simulink model "Prey_Predator_STM32F4"  (R2025a)
settings: Solver=FixedStepDiscrete  StartTime=0.0  StopTime=10.0  RelTol=1e-3
PreLoadFcn:
  | waijung.modelPreload; % Required for working with Waijung Blockset. Do not remove.
undefined symbols (not defined in the file): HSEOSC, Link, LQFP176, ST, STM32F417IG
libraries: stm32f4_io_lib x144, fuzblock x1, stm32f4_device_config_lib x1
(part 2 of 3)

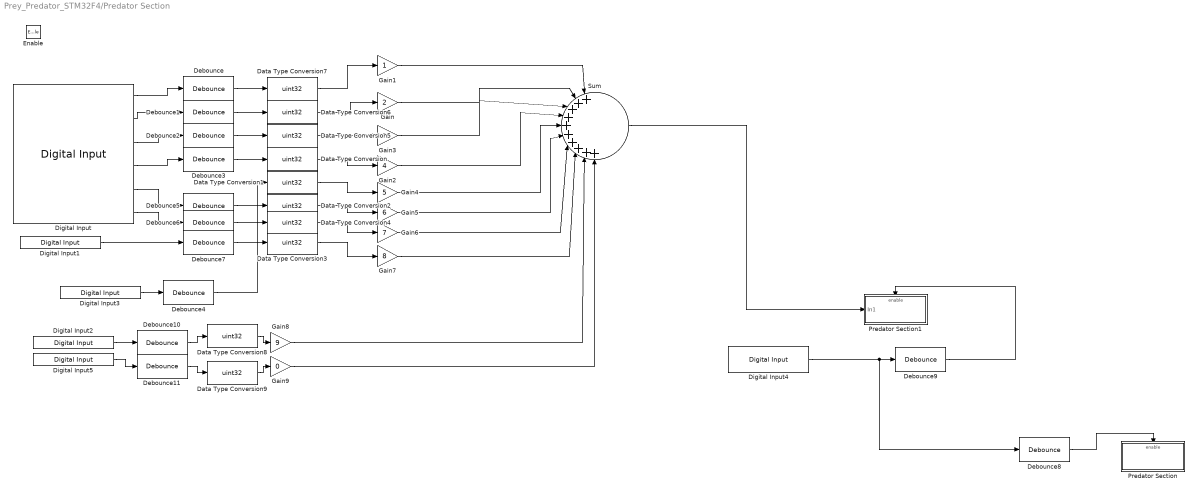
== system Prey_Predator_STM32F4/Predator Section ==
  Enable : EnablePort  PropagateVarSize=During execution
  Data Type Conversion{,1..9} (10 alike) : DataTypeConversion  OutDataTypeStr=uint32  SaturateOnIntegerOverflow=off  RndMeth=Floor
  Debounce{,1..8,10..11} (11 alike) : stm32f4_io_lib/Debounce  mode=Normal  prescale=4  debounce=4
      settings: SourceProductName=IO
  Debounce9 : stm32f4_io_lib/Debounce  mode=Single Pulse  prescale=4  debounce=4
      settings: SourceProductName=IO
  Digital Input : stm32f4_io_lib/Digital Input  port=D  speed=100  porttype=None  porttypestr=NOPULL  use_pin0=off  use_pin1=on  use_pin2=on  use_pin3=on  use_pin4=on  use_pin5=off  use_pin6=on  use_pin7=on  use_pin8=off  use_pin9=off  use_pin10=off  use_pin11=off  use_pin12=off  use_pin13=off  use_pin14=off  use_pin15=off  pinstr=GPIO_Pin_1 | GPIO_Pin_2 | GPIO_Pin_3 | GPIO_Pin_4 | GPIO_Pin_6 | GPIO_Pin_7  usedpinarray="[0  1  1  1  1  0  1  1  0  0  0  0  0  0  0  0]"  bitbandingstr=|  sampletime=0.01  sampletimestr=-1  blockid=PredatorSectionDigitalInput  enablecustomportlabel=off  glabalinit=off  cinputportlabel=In1, In2  coutputportlabel=Out1, Out2
      | #define PredatorSectionDigitalInput_D1 Peripheral_BB(GPIOD->IDR, 1)  /* Output pin */
      | #define PredatorSectionDigitalInput_D2 Peripheral_BB(GPIOD->IDR, 2)  /* Output pin */
      | #define PredatorSectionDigitalInput_D3 Peripheral_BB(GPIOD->IDR, 3)  /* Output pin */
      | #define PredatorSectionDigitalInput_D4 Peripheral_BB(GPIOD->IDR, 4)  /* Output pin */
      | #define PredatorSectionDigitalInput_D6 Peripheral_BB(GPIOD->IDR, 6)  /* Output pin */
      | #define PredatorSectionDigitalInput_D7 Peripheral_BB(GPIOD->IDR, 7)  /* Output pin */
      settings: SourceProductName=IO
  Digital Input1 : stm32f4_io_lib/Digital Input  port=B  speed=100  porttype=None  porttypestr=NOPULL  use_pin0=off  use_pin1=off  use_pin2=off  use_pin3=on  use_pin4=off  use_pin5=off  use_pin6=off  use_pin7=off  use_pin8=off  use_pin9=off  use_pin10=off  use_pin11=off  use_pin12=off  use_pin13=off  use_pin14=off  use_pin15=off  pinstr=GPIO_Pin_3  usedpinarray="[0  0  0  1  0  0  0  0  0  0  0  0  0  0  0  0]"  bitbandingstr="#define PredatorSectionDigitalInput1_B3 Peripheral_BB(GPIOB->IDR, 3)  /* Output pin */"  sampletime=0.01  sampletimestr=-1  blockid=PredatorSectionDigitalInput1  enablecustomportlabel=off  glabalinit=off  cinputportlabel=In1, In2  coutputportlabel=Out1, Out2
      settings: SourceProductName=IO
  Digital Input2 : stm32f4_io_lib/Digital Input  port=A  speed=100  porttype=None  porttypestr=NOPULL  use_pin0=off  use_pin1=on  use_pin2=off  use_pin3=off  use_pin4=off  use_pin5=off  use_pin6=off  use_pin7=off  use_pin8=off  use_pin9=off  use_pin10=off  use_pin11=off  use_pin12=off  use_pin13=off  use_pin14=off  use_pin15=off  pinstr=GPIO_Pin_1  usedpinarray="[0  1  0  0  0  0  0  0  0  0  0  0  0  0  0  0]"  bitbandingstr="#define PredatorSectionDigitalInput2_A1 Peripheral_BB(GPIOA->IDR, 1)  /* Output pin */"  sampletime=0.01  sampletimestr=-1  blockid=PredatorSectionDigitalInput2  enablecustomportlabel=off  glabalinit=off  cinputportlabel=In1, In2  coutputportlabel=Out1, Out2
      settings: SourceProductName=IO
  Digital Input3 : stm32f4_io_lib/Digital Input  port=B  speed=100  porttype=None  porttypestr=NOPULL  use_pin0=off  use_pin1=off  use_pin2=off  use_pin3=off  use_pin4=off  use_pin5=on  use_pin6=off  use_pin7=off  use_pin8=off  use_pin9=off  use_pin10=off  use_pin11=off  use_pin12=off  use_pin13=off  use_pin14=off  use_pin15=off  pinstr=GPIO_Pin_5  usedpinarray="[0  0  0  0  0  1  0  0  0  0  0  0  0  0  0  0]"  bitbandingstr="#define PredatorSectionDigitalInput3_B5 Peripheral_BB(GPIOB->IDR, 5)  /* Output pin */"  sampletime=0.01  sampletimestr=-1  blockid=PredatorSectionDigitalInput3  enablecustomportlabel=off  glabalinit=off  cinputportlabel=In1, In2  coutputportlabel=Out1, Out2
      settings: SourceProductName=IO
  Digital Input4 : stm32f4_io_lib/Digital Input  port=E  speed=100  porttype=None  porttypestr=NOPULL  use_pin0=off  use_pin1=off  use_pin2=on  use_pin3=off  use_pin4=off  use_pin5=off  use_pin6=off  use_pin7=off  use_pin8=off  use_pin9=off  use_pin10=off  use_pin11=off  use_pin12=off  use_pin13=off  use_pin14=off  use_pin15=off  pinstr=GPIO_Pin_2  usedpinarray="[0  0  1  0  0  0  0  0  0  0  0  0  0  0  0  0]"  bitbandingstr="#define PredatorSectionDigitalInput4_E2 Peripheral_BB(GPIOE->IDR, 2)  /* Output pin */"  sampletime=0.01  sampletimestr=-1  blockid=PredatorSectionDigitalInput4  enablecustomportlabel=off  glabalinit=off  cinputportlabel=In1, In2  coutputportlabel=Out1, Out2
      settings: SourceProductName=IO
  Digital Input5 : stm32f4_io_lib/Digital Input  port=A  speed=100  porttype=None  porttypestr=NOPULL  use_pin0=on  use_pin1=off  use_pin2=off  use_pin3=off  use_pin4=off  use_pin5=off  use_pin6=off  use_pin7=off  use_pin8=off  use_pin9=off  use_pin10=off  use_pin11=off  use_pin12=off  use_pin13=off  use_pin14=off  use_pin15=off  pinstr=GPIO_Pin_0  usedpinarray="[1  0  0  0  0  0  0  0  0  0  0  0  0  0  0  0]"  bitbandingstr="#define PredatorSectionDigitalInput5_A0 Peripheral_BB(GPIOA->IDR, 0)  /* Output pin */"  sampletime=0.01  sampletimestr=-1  blockid=PredatorSectionDigitalInput5  enablecustomportlabel=off  glabalinit=off  cinputportlabel=In1, In2  coutputportlabel=Out1, Out2
      settings: SourceProductName=IO
  Gain : Gain  Gain=2  OutDataTypeStr=Inherit: Same as input
  Gain1 : Gain  OutDataTypeStr=Inherit: Same as input
  Gain2 : Gain  Gain=4  OutDataTypeStr=Inherit: Same as input
  Gain3 : Gain  Gain=3  OutDataTypeStr=Inherit: Same as input
  Gain4 : Gain  Gain=5  OutDataTypeStr=Inherit: Same as input
  Gain5 : Gain  Gain=6  OutDataTypeStr=Inherit: Same as input
  Gain6 : Gain  Gain=7  OutDataTypeStr=Inherit: Same as input
  Gain7 : Gain  Gain=8  OutDataTypeStr=Inherit: Same as input
  Gain8 : Gain  Gain=9  OutDataTypeStr=Inherit: Same as input
  Gain9 : Gain  Gain=0  OutDataTypeStr=Inherit: Same as input
  Predator Section : Subsystem
  Predator Section1 : Subsystem
  Sum : Sum  Inputs=|++++++++++
  wires:
  Digital Input/4 -> Debounce3/1
  Digital Input/3 -> Debounce2/1
  Digital Input/2 -> Debounce1/1
  Digital Input/1 -> Debounce/1
  Digital Input1/1 -> Debounce7/1
  Debounce/1 -> Data Type Conversion7/1
  Debounce1/1 -> Data Type Conversion6/1
  Debounce2/1 -> Data Type Conversion5/1
  Debounce3/1 -> Data Type Conversion/1
  Debounce4/1 -> Data Type Conversion1/1
  Debounce5/1 -> Data Type Conversion2/1
  Debounce6/1 -> Data Type Conversion4/1
  Debounce7/1 -> Data Type Conversion3/1
  Data Type Conversion7/1 -> Gain1/1
  Data Type Conversion6/1 -> Gain/1
  Data Type Conversion5/1 -> Gain3/1
  Data Type Conversion/1 -> Gain2/1
  Data Type Conversion1/1 -> Gain4/1
  Data Type Conversion2/1 -> Gain5/1
  Data Type Conversion4/1 -> Gain6/1
  Data Type Conversion3/1 -> Gain7/1
  Gain1/1 -> Sum/1
  Gain/1 -> Sum/2
  Gain3/1 -> Sum/3
  Gain2/1 -> Sum/4
  Gain4/1 -> Sum/5
  Gain5/1 -> Sum/6
  Gain6/1 -> Sum/7
  Gain7/1 -> Sum/8
  Digital Input/5 -> Debounce5/1
  Digital Input/6 -> Debounce6/1
  Digital Input3/1 -> Debounce4/1
  Sum/1 -> Predator Section1/1(In1)
  Digital Input4/1 -> Debounce8/1, Debounce9/1
  Debounce9/1 -> Predator Section1/Enable
  Debounce8/1 -> Predator Section/Enable
  Digital Input2/1 -> Debounce10/1
  Digital Input5/1 -> Debounce11/1
  Debounce11/1 -> Data Type Conversion9/1
  Debounce10/1 -> Data Type Conversion8/1
  Data Type Conversion8/1 -> Gain8/1
  Data Type Conversion9/1 -> Gain9/1
  Gain8/1 -> Sum/9
  Gain9/1 -> Sum/10

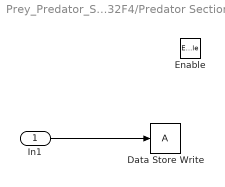
== system Prey_Predator_STM32F4/Predator Section1 ==
  In1 : Inport
  Enable : EnablePort  PropagateVarSize=During execution
  Data Store Write : DataStoreWrite  IndexOptions=Index vector (dialog)  Indices=1  OutputSizes=1
  wires:
  In1/1 -> Data Store Write/1

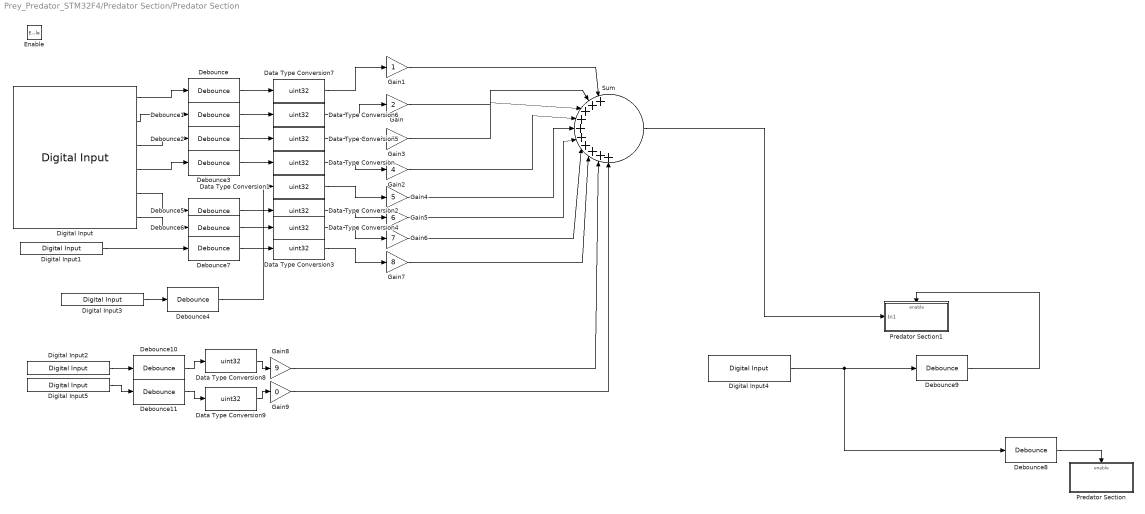
== system Prey_Predator_STM32F4/Predator Section/Predator Section ==
  Enable : EnablePort  PropagateVarSize=During execution
  Data Type Conversion{,1..9} (10 alike) : DataTypeConversion  OutDataTypeStr=uint32  SaturateOnIntegerOverflow=off  RndMeth=Floor
  Debounce{,1..8,10..11} (11 alike) : stm32f4_io_lib/Debounce  mode=Normal  prescale=4  debounce=4
      settings: SourceProductName=IO
  Debounce9 : stm32f4_io_lib/Debounce  mode=Single Pulse  prescale=4  debounce=4
      settings: SourceProductName=IO
  Digital Input : stm32f4_io_lib/Digital Input  port=D  speed=100  porttype=None  porttypestr=NOPULL  use_pin0=off  use_pin1=on  use_pin2=on  use_pin3=on  use_pin4=on  use_pin5=off  use_pin6=on  use_pin7=on  use_pin8=off  use_pin9=off  use_pin10=off  use_pin11=off  use_pin12=off  use_pin13=off  use_pin14=off  use_pin15=off  pinstr=GPIO_Pin_1 | GPIO_Pin_2 | GPIO_Pin_3 | GPIO_Pin_4 | GPIO_Pin_6 | GPIO_Pin_7  usedpinarray="[0  1  1  1  1  0  1  1  0  0  0  0  0  0  0  0]"  bitbandingstr=|  sampletime=0.01  sampletimestr=-1  blockid=PredatorSectionPredatorSectionDigitalInput  enablecustomportlabel=off  glabalinit=off  cinputportlabel=In1, In2  coutputportlabel=Out1, Out2
      | #define PredatorSectionPredatorSectionDigitalInput_D1 Peripheral_BB(GPIOD->IDR, 1)  /* Output pin */
      | #define PredatorSectionPredatorSectionDigitalInput_D2 Peripheral_BB(GPIOD->IDR, 2)  /* Output pin */
      | #define PredatorSectionPredatorSectionDigitalInput_D3 Peripheral_BB(GPIOD->IDR, 3)  /* Output pin */
      | #define PredatorSectionPredatorSectionDigitalInput_D4 Peripheral_BB(GPIOD->IDR, 4)  /* Output pin */
      | #define PredatorSectionPredatorSectionDigitalInput_D6 Peripheral_BB(GPIOD->IDR, 6)  /* Output pin */
      | #define PredatorSectionPredatorSectionDigitalInput_D7 Peripheral_BB(GPIOD->IDR, 7)  /* Output pin */
      settings: SourceProductName=IO
  Digital Input1 : stm32f4_io_lib/Digital Input  port=B  speed=100  porttype=None  porttypestr=NOPULL  use_pin0=off  use_pin1=off  use_pin2=off  use_pin3=on  use_pin4=off  use_pin5=off  use_pin6=off  use_pin7=off  use_pin8=off  use_pin9=off  use_pin10=off  use_pin11=off  use_pin12=off  use_pin13=off  use_pin14=off  use_pin15=off  pinstr=GPIO_Pin_3  usedpinarray="[0  0  0  1  0  0  0  0  0  0  0  0  0  0  0  0]"  bitbandingstr="#define PredatorSectionPredatorSectionDigitalInput1_B3 Peripheral_BB(GPIOB->IDR, 3)  /* Output pin */"  sampletime=0.01  sampletimestr=-1  blockid=PredatorSectionPredatorSectionDigitalInput1  enablecustomportlabel=off  glabalinit=off  cinputportlabel=In1, In2  coutputportlabel=Out1, Out2
      settings: SourceProductName=IO
  Digital Input2 : stm32f4_io_lib/Digital Input  port=A  speed=100  porttype=None  porttypestr=NOPULL  use_pin0=off  use_pin1=on  use_pin2=off  use_pin3=off  use_pin4=off  use_pin5=off  use_pin6=off  use_pin7=off  use_pin8=off  use_pin9=off  use_pin10=off  use_pin11=off  use_pin12=off  use_pin13=off  use_pin14=off  use_pin15=off  pinstr=GPIO_Pin_1  usedpinarray="[0  1  0  0  0  0  0  0  0  0  0  0  0  0  0  0]"  bitbandingstr="#define PredatorSectionPredatorSectionDigitalInput2_A1 Peripheral_BB(GPIOA->IDR, 1)  /* Output pin */"  sampletime=0.01  sampletimestr=-1  blockid=PredatorSectionPredatorSectionDigitalInput2  enablecustomportlabel=off  glabalinit=off  cinputportlabel=In1, In2  coutputportlabel=Out1, Out2
      settings: SourceProductName=IO
  Digital Input3 : stm32f4_io_lib/Digital Input  port=B  speed=100  porttype=None  porttypestr=NOPULL  use_pin0=off  use_pin1=off  use_pin2=off  use_pin3=off  use_pin4=off  use_pin5=on  use_pin6=off  use_pin7=off  use_pin8=off  use_pin9=off  use_pin10=off  use_pin11=off  use_pin12=off  use_pin13=off  use_pin14=off  use_pin15=off  pinstr=GPIO_Pin_5  usedpinarray="[0  0  0  0  0  1  0  0  0  0  0  0  0  0  0  0]"  bitbandingstr="#define PredatorSectionPredatorSectionDigitalInput3_B5 Peripheral_BB(GPIOB->IDR, 5)  /* Output pin */"  sampletime=0.01  sampletimestr=-1  blockid=PredatorSectionPredatorSectionDigitalInput3  enablecustomportlabel=off  glabalinit=off  cinputportlabel=In1, In2  coutputportlabel=Out1, Out2
      settings: SourceProductName=IO
  Digital Input4 : stm32f4_io_lib/Digital Input  port=A  speed=100  porttype=None  porttypestr=NOPULL  use_pin0=off  use_pin1=off  use_pin2=off  use_pin3=off  use_pin4=off  use_pin5=off  use_pin6=off  use_pin7=off  use_pin8=off  use_pin9=off  use_pin10=off  use_pin11=off  use_pin12=off  use_pin13=off  use_pin14=off  use_pin15=on  pinstr=GPIO_Pin_15  usedpinarray="[0  0  0  0  0  0  0  0  0  0  0  0  0  0  0  1]"  bitbandingstr="#define PredatorSectionPredatorSectionDigitalInput4_A15 Peripheral_BB(GPIOA->IDR, 15)  /* Output pin */"  sampletime=0.01  sampletimestr=-1  blockid=PredatorSectionPredatorSectionDigitalInput4  enablecustomportlabel=off  glabalinit=off  cinputportlabel=In1, In2  coutputportlabel=Out1, Out2
      settings: SourceProductName=IO
  Digital Input5 : stm32f4_io_lib/Digital Input  port=A  speed=100  porttype=None  porttypestr=NOPULL  use_pin0=on  use_pin1=off  use_pin2=off  use_pin3=off  use_pin4=off  use_pin5=off  use_pin6=off  use_pin7=off  use_pin8=off  use_pin9=off  use_pin10=off  use_pin11=off  use_pin12=off  use_pin13=off  use_pin14=off  use_pin15=off  pinstr=GPIO_Pin_0  usedpinarray="[1  0  0  0  0  0  0  0  0  0  0  0  0  0  0  0]"  bitbandingstr="#define PredatorSectionPredatorSectionDigitalInput5_A0 Peripheral_BB(GPIOA->IDR, 0)  /* Output pin */"  sampletime=0.01  sampletimestr=-1  blockid=PredatorSectionPredatorSectionDigitalInput5  enablecustomportlabel=off  glabalinit=off  cinputportlabel=In1, In2  coutputportlabel=Out1, Out2
      settings: SourceProductName=IO
  Gain : Gain  Gain=2  OutDataTypeStr=Inherit: Same as input
  Gain1 : Gain  OutDataTypeStr=Inherit: Same as input
  Gain2 : Gain  Gain=4  OutDataTypeStr=Inherit: Same as input
  Gain3 : Gain  Gain=3  OutDataTypeStr=Inherit: Same as input
  Gain4 : Gain  Gain=5  OutDataTypeStr=Inherit: Same as input
  Gain5 : Gain  Gain=6  OutDataTypeStr=Inherit: Same as input
  Gain6 : Gain  Gain=7  OutDataTypeStr=Inherit: Same as input
  Gain7 : Gain  Gain=8  OutDataTypeStr=Inherit: Same as input
  Gain8 : Gain  Gain=9  OutDataTypeStr=Inherit: Same as input
  Gain9 : Gain  Gain=0  OutDataTypeStr=Inherit: Same as input
  Predator Section : Subsystem
  Predator Section1 : Subsystem
  Sum : Sum  Inputs=|++++++++++
  wires:
  Digital Input/4 -> Debounce3/1
  Digital Input/3 -> Debounce2/1
  Digital Input/2 -> Debounce1/1
  Digital Input/1 -> Debounce/1
  Digital Input1/1 -> Debounce7/1
  Debounce/1 -> Data Type Conversion7/1
  Debounce1/1 -> Data Type Conversion6/1
  Debounce2/1 -> Data Type Conversion5/1
  Debounce3/1 -> Data Type Conversion/1
  Debounce4/1 -> Data Type Conversion1/1
  Debounce5/1 -> Data Type Conversion2/1
  Debounce6/1 -> Data Type Conversion4/1
  Debounce7/1 -> Data Type Conversion3/1
  Data Type Conversion7/1 -> Gain1/1
  Data Type Conversion6/1 -> Gain/1
  Data Type Conversion5/1 -> Gain3/1
  Data Type Conversion/1 -> Gain2/1
  Data Type Conversion1/1 -> Gain4/1
  Data Type Conversion2/1 -> Gain5/1
  Data Type Conversion4/1 -> Gain6/1
  Data Type Conversion3/1 -> Gain7/1
  Gain1/1 -> Sum/1
  Gain/1 -> Sum/2
  Gain3/1 -> Sum/3
  Gain2/1 -> Sum/4
  Gain4/1 -> Sum/5
  Gain5/1 -> Sum/6
  Gain6/1 -> Sum/7
  Gain7/1 -> Sum/8
  Digital Input/5 -> Debounce5/1
  Digital Input/6 -> Debounce6/1
  Digital Input3/1 -> Debounce4/1
  Sum/1 -> Predator Section1/1(In1)
  Digital Input4/1 -> Debounce8/1, Debounce9/1
  Debounce9/1 -> Predator Section1/Enable
  Debounce8/1 -> Predator Section/Enable
  Digital Input2/1 -> Debounce10/1
  Digital Input5/1 -> Debounce11/1
  Debounce11/1 -> Data Type Conversion9/1
  Debounce10/1 -> Data Type Conversion8/1
  Data Type Conversion8/1 -> Gain8/1
  Data Type Conversion9/1 -> Gain9/1
  Gain8/1 -> Sum/9
  Gain9/1 -> Sum/10

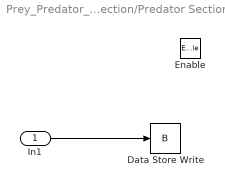
== system Prey_Predator_STM32F4/Predator Section/Predator Section1 ==
  In1 : Inport
  Enable : EnablePort  PropagateVarSize=During execution
  Data Store Write : DataStoreWrite  DataStoreName=B  IndexOptions=Index vector (dialog)  Indices=1  OutputSizes=1
  wires:
  In1/1 -> Data Store Write/1

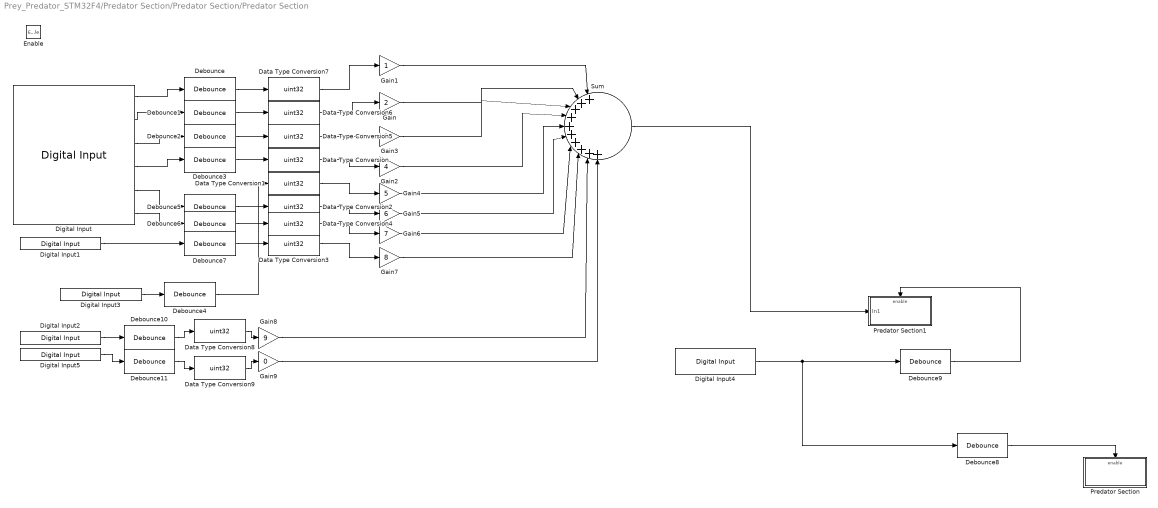
== system Prey_Predator_STM32F4/Predator Section/Predator Section/Predator Section ==
  Enable : EnablePort  PropagateVarSize=During execution
  Data Type Conversion{,1..9} (10 alike) : DataTypeConversion  OutDataTypeStr=uint32  SaturateOnIntegerOverflow=off  RndMeth=Floor
  Debounce{,1..8,10..11} (11 alike) : stm32f4_io_lib/Debounce  mode=Normal  prescale=4  debounce=4
      settings: SourceProductName=IO
  Debounce9 : stm32f4_io_lib/Debounce  mode=Single Pulse  prescale=4  debounce=4
      settings: SourceProductName=IO
  Digital Input : stm32f4_io_lib/Digital Input  port=D  speed=100  porttype=None  porttypestr=NOPULL  use_pin0=off  use_pin1=on  use_pin2=on  use_pin3=on  use_pin4=on  use_pin5=off  use_pin6=on  use_pin7=on  use_pin8=off  use_pin9=off  use_pin10=off  use_pin11=off  use_pin12=off  use_pin13=off  use_pin14=off  use_pin15=off  pinstr=GPIO_Pin_1 | GPIO_Pin_2 | GPIO_Pin_3 | GPIO_Pin_4 | GPIO_Pin_6 | GPIO_Pin_7  usedpinarray="[0  1  1  1  1  0  1  1  0  0  0  0  0  0  0  0]"  bitbandingstr=|  sampletime=0.01  sampletimestr=-1  blockid=PredatorSectionPredatorSectionPredatorSectionDigitalInput  enablecustomportlabel=off  glabalinit=off  cinputportlabel=In1, In2  coutputportlabel=Out1, Out2
      | #define PredatorSectionPredatorSectionPredatorSectionDigitalInput_D1 Peripheral_BB(GPIOD->IDR, 1)  /* Output pin */
      | #define PredatorSectionPredatorSectionPredatorSectionDigitalInput_D2 Peripheral_BB(GPIOD->IDR, 2)  /* Output pin */
      | #define PredatorSectionPredatorSectionPredatorSectionDigitalInput_D3 Peripheral_BB(GPIOD->IDR, 3)  /* Output pin */
      | #define PredatorSectionPredatorSectionPredatorSectionDigitalInput_D4 Peripheral_BB(GPIOD->IDR, 4)  /* Output pin */
      | #define PredatorSectionPredatorSectionPredatorSectionDigitalInput_D6 Peripheral_BB(GPIOD->IDR, 6)  /* Output pin */
      | #define PredatorSectionPredatorSectionPredatorSectionDigitalInput_D7 Peripheral_BB(GPIOD->IDR, 7)  /* Output pin */
      settings: SourceProductName=IO
  Digital Input1 : stm32f4_io_lib/Digital Input  port=B  speed=100  porttype=None  porttypestr=NOPULL  use_pin0=off  use_pin1=off  use_pin2=off  use_pin3=on  use_pin4=off  use_pin5=off  use_pin6=off  use_pin7=off  use_pin8=off  use_pin9=off  use_pin10=off  use_pin11=off  use_pin12=off  use_pin13=off  use_pin14=off  use_pin15=off  pinstr=GPIO_Pin_3  usedpinarray="[0  0  0  1  0  0  0  0  0  0  0  0  0  0  0  0]"  bitbandingstr="#define PredatorSectionPredatorSectionPredatorSectionDigitalInput1_B3 Peripheral_BB(GPIOB->IDR, 3)  /* Output pin */"  sampletime=0.01  sampletimestr=-1  blockid=PredatorSectionPredatorSectionPredatorSectionDigitalInput1  enablecustomportlabel=off  glabalinit=off  cinputportlabel=In1, In2  coutputportlabel=Out1, Out2
      settings: SourceProductName=IO
  Digital Input2 : stm32f4_io_lib/Digital Input  port=A  speed=100  porttype=None  porttypestr=NOPULL  use_pin0=off  use_pin1=on  use_pin2=off  use_pin3=off  use_pin4=off  use_pin5=off  use_pin6=off  use_pin7=off  use_pin8=off  use_pin9=off  use_pin10=off  use_pin11=off  use_pin12=off  use_pin13=off  use_pin14=off  use_pin15=off  pinstr=GPIO_Pin_1  usedpinarray="[0  1  0  0  0  0  0  0  0  0  0  0  0  0  0  0]"  bitbandingstr="#define PredatorSectionPredatorSectionPredatorSectionDigitalInput2_A1 Peripheral_BB(GPIOA->IDR, 1)  /* Output pin */"  sampletime=0.01  sampletimestr=-1  blockid=PredatorSectionPredatorSectionPredatorSectionDigitalInput2  enablecustomportlabel=off  glabalinit=off  cinputportlabel=In1, In2  coutputportlabel=Out1, Out2
      settings: SourceProductName=IO
  Digital Input3 : stm32f4_io_lib/Digital Input  port=B  speed=100  porttype=None  porttypestr=NOPULL  use_pin0=off  use_pin1=off  use_pin2=off  use_pin3=off  use_pin4=off  use_pin5=on  use_pin6=off  use_pin7=off  use_pin8=off  use_pin9=off  use_pin10=off  use_pin11=off  use_pin12=off  use_pin13=off  use_pin14=off  use_pin15=off  pinstr=GPIO_Pin_5  usedpinarray="[0  0  0  0  0  1  0  0  0  0  0  0  0  0  0  0]"  bitbandingstr="#define PredatorSectionPredatorSectionPredatorSectionDigitalInput3_B5 Peripheral_BB(GPIOB->IDR, 5)  /* Output pin */"  sampletime=0.01  sampletimestr=-1  blockid=PredatorSectionPredatorSectionPredatorSectionDigitalInput3  enablecustomportlabel=off  glabalinit=off  cinputportlabel=In1, In2  coutputportlabel=Out1, Out2
      settings: SourceProductName=IO
  Digital Input4 : stm32f4_io_lib/Digital Input  port=E  speed=100  porttype=None  porttypestr=NOPULL  use_pin0=off  use_pin1=off  use_pin2=off  use_pin3=off  use_pin4=on  use_pin5=off  use_pin6=off  use_pin7=off  use_pin8=off  use_pin9=off  use_pin10=off  use_pin11=off  use_pin12=off  use_pin13=off  use_pin14=off  use_pin15=off  pinstr=GPIO_Pin_4  usedpinarray="[0  0  0  0  1  0  0  0  0  0  0  0  0  0  0  0]"  bitbandingstr="#define PredatorSectionPredatorSectionPredatorSectionDigitalInput4_E4 Peripheral_BB(GPIOE->IDR, 4)  /* Output pin */"  sampletime=0.01  sampletimestr=-1  blockid=PredatorSectionPredatorSectionPredatorSectionDigitalInput4  enablecustomportlabel=off  glabalinit=off  cinputportlabel=In1, In2  coutputportlabel=Out1, Out2
      settings: SourceProductName=IO
  Digital Input5 : stm32f4_io_lib/Digital Input  port=A  speed=100  porttype=None  porttypestr=NOPULL  use_pin0=on  use_pin1=off  use_pin2=off  use_pin3=off  use_pin4=off  use_pin5=off  use_pin6=off  use_pin7=off  use_pin8=off  use_pin9=off  use_pin10=off  use_pin11=off  use_pin12=off  use_pin13=off  use_pin14=off  use_pin15=off  pinstr=GPIO_Pin_0  usedpinarray="[1  0  0  0  0  0  0  0  0  0  0  0  0  0  0  0]"  bitbandingstr="#define PredatorSectionPredatorSectionPredatorSectionDigitalInput5_A0 Peripheral_BB(GPIOA->IDR, 0)  /* Output pin */"  sampletime=0.01  sampletimestr=-1  blockid=PredatorSectionPredatorSectionPredatorSectionDigitalInput5  enablecustomportlabel=off  glabalinit=off  cinputportlabel=In1, In2  coutputportlabel=Out1, Out2
      settings: SourceProductName=IO
  Gain : Gain  Gain=2  OutDataTypeStr=Inherit: Same as input
  Gain1 : Gain  OutDataTypeStr=Inherit: Same as input
  Gain2 : Gain  Gain=4  OutDataTypeStr=Inherit: Same as input
  Gain3 : Gain  Gain=3  OutDataTypeStr=Inherit: Same as input
  Gain4 : Gain  Gain=5  OutDataTypeStr=Inherit: Same as input
  Gain5 : Gain  Gain=6  OutDataTypeStr=Inherit: Same as input
  Gain6 : Gain  Gain=7  OutDataTypeStr=Inherit: Same as input
  Gain7 : Gain  Gain=8  OutDataTypeStr=Inherit: Same as input
  Gain8 : Gain  Gain=9  OutDataTypeStr=Inherit: Same as input
  Gain9 : Gain  Gain=0  OutDataTypeStr=Inherit: Same as input
  Predator Section : Subsystem
  Predator Section1 : Subsystem
  Sum : Sum  Inputs=|++++++++++
  wires:
  Digital Input/4 -> Debounce3/1
  Digital Input/3 -> Debounce2/1
  Digital Input/2 -> Debounce1/1
  Digital Input/1 -> Debounce/1
  Digital Input1/1 -> Debounce7/1
  Debounce/1 -> Data Type Conversion7/1
  Debounce1/1 -> Data Type Conversion6/1
  Debounce2/1 -> Data Type Conversion5/1
  Debounce3/1 -> Data Type Conversion/1
  Debounce4/1 -> Data Type Conversion1/1
  Debounce5/1 -> Data Type Conversion2/1
  Debounce6/1 -> Data Type Conversion4/1
  Debounce7/1 -> Data Type Conversion3/1
  Data Type Conversion7/1 -> Gain1/1
  Data Type Conversion6/1 -> Gain/1
  Data Type Conversion5/1 -> Gain3/1
  Data Type Conversion/1 -> Gain2/1
  Data Type Conversion1/1 -> Gain4/1
  Data Type Conversion2/1 -> Gain5/1
  Data Type Conversion4/1 -> Gain6/1
  Data Type Conversion3/1 -> Gain7/1
  Gain1/1 -> Sum/1
  Gain/1 -> Sum/2
  Gain3/1 -> Sum/3
  Gain2/1 -> Sum/4
  Gain4/1 -> Sum/5
  Gain5/1 -> Sum/6
  Gain6/1 -> Sum/7
  Gain7/1 -> Sum/8
  Digital Input/5 -> Debounce5/1
  Digital Input/6 -> Debounce6/1
  Digital Input3/1 -> Debounce4/1
  Sum/1 -> Predator Section1/1(In1)
  Digital Input4/1 -> Debounce8/1, Debounce9/1
  Debounce9/1 -> Predator Section1/Enable
  Debounce8/1 -> Predator Section/Enable
  Digital Input2/1 -> Debounce10/1
  Digital Input5/1 -> Debounce11/1
  Debounce11/1 -> Data Type Conversion9/1
  Debounce10/1 -> Data Type Conversion8/1
  Data Type Conversion8/1 -> Gain8/1
  Data Type Conversion9/1 -> Gain9/1
  Gain8/1 -> Sum/9
  Gain9/1 -> Sum/10

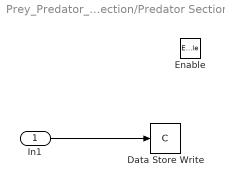
== system Prey_Predator_STM32F4/Predator Section/Predator Section/Predator Section1 ==
  In1 : Inport
  Enable : EnablePort  PropagateVarSize=During execution
  Data Store Write : DataStoreWrite  DataStoreName=C  IndexOptions=Index vector (dialog)  Indices=1  OutputSizes=1
  wires:
  In1/1 -> Data Store Write/1

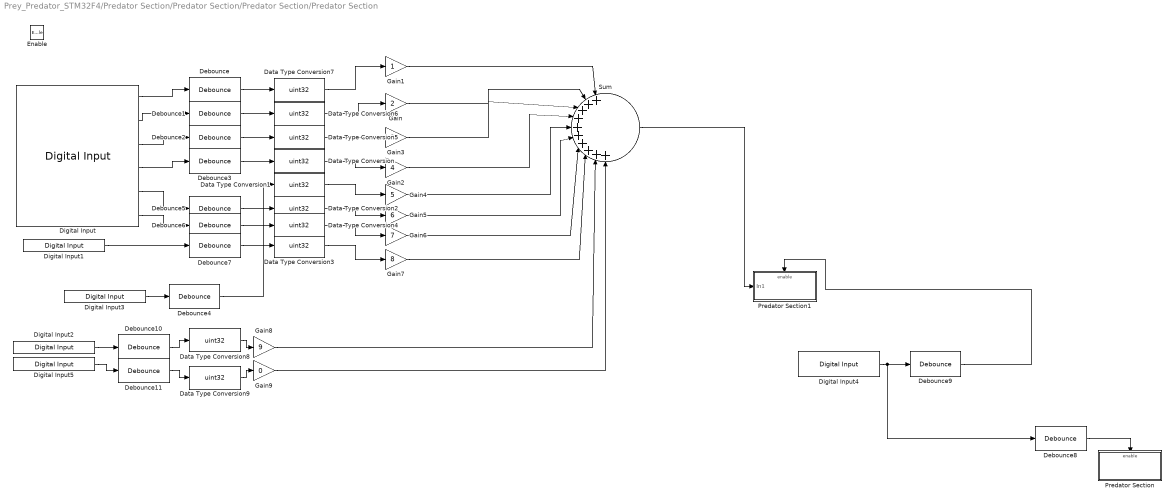
== system Prey_Predator_STM32F4/Predator Section/Predator Section/Predator Section/Predator Section ==
  Enable : EnablePort  PropagateVarSize=During execution
  Data Type Conversion{,1..9} (10 alike) : DataTypeConversion  OutDataTypeStr=uint32  SaturateOnIntegerOverflow=off  RndMeth=Floor
  Debounce{,1..8,10..11} (11 alike) : stm32f4_io_lib/Debounce  mode=Normal  prescale=4  debounce=4
      settings: SourceProductName=IO
  Debounce9 : stm32f4_io_lib/Debounce  mode=Single Pulse  prescale=4  debounce=4
      settings: SourceProductName=IO
  Digital Input : stm32f4_io_lib/Digital Input  port=D  speed=100  porttype=None  porttypestr=NOPULL  use_pin0=off  use_pin1=on  use_pin2=on  use_pin3=on  use_pin4=on  use_pin5=off  use_pin6=on  use_pin7=on  use_pin8=off  use_pin9=off  use_pin10=off  use_pin11=off  use_pin12=off  use_pin13=off  use_pin14=off  use_pin15=off  pinstr=GPIO_Pin_1 | GPIO_Pin_2 | GPIO_Pin_3 | GPIO_Pin_4 | GPIO_Pin_6 | GPIO_Pin_7  usedpinarray="[0  1  1  1  1  0  1  1  0  0  0  0  0  0  0  0]"  bitbandingstr=|  sampletime=0.01  sampletimestr=-1  blockid=PredatorSectionPredatorSectionPredatorSectionPredatorSectionDigitalInput  enablecustomportlabel=off  glabalinit=off  cinputportlabel=In1, In2  coutputportlabel=Out1, Out2
      | #define PredatorSectionPredatorSectionPredatorSectionPredatorSectionDigitalInput_D1 Peripheral_BB(GPIOD->IDR, 1)  /* Output pin */
      | #define PredatorSectionPredatorSectionPredatorSectionPredatorSectionDigitalInput_D2 Peripheral_BB(GPIOD->IDR, 2)  /* Output pin */
      | #define PredatorSectionPredatorSectionPredatorSectionPredatorSectionDigitalInput_D3 Peripheral_BB(GPIOD->IDR, 3)  /* Output pin */
      | #define PredatorSectionPredatorSectionPredatorSectionPredatorSectionDigitalInput_D4 Peripheral_BB(GPIOD->IDR, 4)  /* Output pin */
      | #define PredatorSectionPredatorSectionPredatorSectionPredatorSectionDigitalInput_D6 Peripheral_BB(GPIOD->IDR, 6)  /* Output pin */
      | #define PredatorSectionPredatorSectionPredatorSectionPredatorSectionDigitalInput_D7 Peripheral_BB(GPIOD->IDR, 7)  /* Output pin */
      settings: SourceProductName=IO
  Digital Input1 : stm32f4_io_lib/Digital Input  port=B  speed=100  porttype=None  porttypestr=NOPULL  use_pin0=off  use_pin1=off  use_pin2=off  use_pin3=on  use_pin4=off  use_pin5=off  use_pin6=off  use_pin7=off  use_pin8=off  use_pin9=off  use_pin10=off  use_pin11=off  use_pin12=off  use_pin13=off  use_pin14=off  use_pin15=off  pinstr=GPIO_Pin_3  usedpinarray="[0  0  0  1  0  0  0  0  0  0  0  0  0  0  0  0]"  bitbandingstr="#define PredatorSectionPredatorSectionPredatorSectionPredatorSectionDigitalInput1_B3 Peripheral_BB(GPIOB->IDR, 3)  /* Output pin */"  sampletime=0.01  sampletimestr=-1  blockid=PredatorSectionPredatorSectionPredatorSectionPredatorSectionDigitalInput1  enablecustomportlabel=off  glabalinit=off  cinputportlabel=In1, In2  coutputportlabel=Out1, Out2
      settings: SourceProductName=IO
  Digital Input2 : stm32f4_io_lib/Digital Input  port=A  speed=100  porttype=None  porttypestr=NOPULL  use_pin0=off  use_pin1=on  use_pin2=off  use_pin3=off  use_pin4=off  use_pin5=off  use_pin6=off  use_pin7=off  use_pin8=off  use_pin9=off  use_pin10=off  use_pin11=off  use_pin12=off  use_pin13=off  use_pin14=off  use_pin15=off  pinstr=GPIO_Pin_1  usedpinarray="[0  1  0  0  0  0  0  0  0  0  0  0  0  0  0  0]"  bitbandingstr="#define PredatorSectionPredatorSectionPredatorSectionPredatorSectionDigitalInput2_A1 Peripheral_BB(GPIOA->IDR, 1)  /* Output pin */"  sampletime=0.01  sampletimestr=-1  blockid=PredatorSectionPredatorSectionPredatorSectionPredatorSectionDigitalInput2  enablecustomportlabel=off  glabalinit=off  cinputportlabel=In1, In2  coutputportlabel=Out1, Out2
      settings: SourceProductName=IO
  Digital Input3 : stm32f4_io_lib/Digital Input  port=B  speed=100  porttype=None  porttypestr=NOPULL  use_pin0=off  use_pin1=off  use_pin2=off  use_pin3=off  use_pin4=off  use_pin5=on  use_pin6=off  use_pin7=off  use_pin8=off  use_pin9=off  use_pin10=off  use_pin11=off  use_pin12=off  use_pin13=off  use_pin14=off  use_pin15=off  pinstr=GPIO_Pin_5  usedpinarray="[0  0  0  0  0  1  0  0  0  0  0  0  0  0  0  0]"  bitbandingstr="#define PredatorSectionPredatorSectionPredatorSectionPredatorSectionDigitalInput3_B5 Peripheral_BB(GPIOB->IDR, 5)  /* Output pin */"  sampletime=0.01  sampletimestr=-1  blockid=PredatorSectionPredatorSectionPredatorSectionPredatorSectionDigitalInput3  enablecustomportlabel=off  glabalinit=off  cinputportlabel=In1, In2  coutputportlabel=Out1, Out2
      settings: SourceProductName=IO
  Digital Input4 : stm32f4_io_lib/Digital Input  port=E  speed=100  porttype=None  porttypestr=NOPULL  use_pin0=off  use_pin1=off  use_pin2=off  use_pin3=off  use_pin4=off  use_pin5=on  use_pin6=off  use_pin7=off  use_pin8=off  use_pin9=off  use_pin10=off  use_pin11=off  use_pin12=off  use_pin13=off  use_pin14=off  use_pin15=off  pinstr=GPIO_Pin_5  usedpinarray="[0  0  0  0  0  1  0  0  0  0  0  0  0  0  0  0]"  bitbandingstr="#define PredatorSectionPredatorSectionPredatorSectionPredatorSectionDigitalInput4_E5 Peripheral_BB(GPIOE->IDR, 5)  /* Output pin */"  sampletime=0.01  sampletimestr=-1  blockid=PredatorSectionPredatorSectionPredatorSectionPredatorSectionDigitalInput4  enablecustomportlabel=off  glabalinit=off  cinputportlabel=In1, In2  coutputportlabel=Out1, Out2
      settings: SourceProductName=IO
  Digital Input5 : stm32f4_io_lib/Digital Input  port=A  speed=100  porttype=None  porttypestr=NOPULL  use_pin0=on  use_pin1=off  use_pin2=off  use_pin3=off  use_pin4=off  use_pin5=off  use_pin6=off  use_pin7=off  use_pin8=off  use_pin9=off  use_pin10=off  use_pin11=off  use_pin12=off  use_pin13=off  use_pin14=off  use_pin15=off  pinstr=GPIO_Pin_0  usedpinarray="[1  0  0  0  0  0  0  0  0  0  0  0  0  0  0  0]"  bitbandingstr="#define PredatorSectionPredatorSectionPredatorSectionPredatorSectionDigitalInput5_A0 Peripheral_BB(GPIOA->IDR, 0)  /* Output pin */"  sampletime=0.01  sampletimestr=-1  blockid=PredatorSectionPredatorSectionPredatorSectionPredatorSectionDigitalInput5  enablecustomportlabel=off  glabalinit=off  cinputportlabel=In1, In2  coutputportlabel=Out1, Out2
      settings: SourceProductName=IO
  Gain : Gain  Gain=2  OutDataTypeStr=Inherit: Same as input
  Gain1 : Gain  OutDataTypeStr=Inherit: Same as input
  Gain2 : Gain  Gain=4  OutDataTypeStr=Inherit: Same as input
  Gain3 : Gain  Gain=3  OutDataTypeStr=Inherit: Same as input
  Gain4 : Gain  Gain=5  OutDataTypeStr=Inherit: Same as input
  Gain5 : Gain  Gain=6  OutDataTypeStr=Inherit: Same as input
  Gain6 : Gain  Gain=7  OutDataTypeStr=Inherit: Same as input
  Gain7 : Gain  Gain=8  OutDataTypeStr=Inherit: Same as input
  Gain8 : Gain  Gain=9  OutDataTypeStr=Inherit: Same as input
  Gain9 : Gain  Gain=0  OutDataTypeStr=Inherit: Same as input
  Predator Section : Subsystem
  Predator Section1 : Subsystem
  Sum : Sum  Inputs=|++++++++++
  wires:
  Digital Input/4 -> Debounce3/1
  Digital Input/3 -> Debounce2/1
  Digital Input/2 -> Debounce1/1
  Digital Input/1 -> Debounce/1
  Digital Input1/1 -> Debounce7/1
  Debounce/1 -> Data Type Conversion7/1
  Debounce1/1 -> Data Type Conversion6/1
  Debounce2/1 -> Data Type Conversion5/1
  Debounce3/1 -> Data Type Conversion/1
  Debounce4/1 -> Data Type Conversion1/1
  Debounce5/1 -> Data Type Conversion2/1
  Debounce6/1 -> Data Type Conversion4/1
  Debounce7/1 -> Data Type Conversion3/1
  Data Type Conversion7/1 -> Gain1/1
  Data Type Conversion6/1 -> Gain/1
  Data Type Conversion5/1 -> Gain3/1
  Data Type Conversion/1 -> Gain2/1
  Data Type Conversion1/1 -> Gain4/1
  Data Type Conversion2/1 -> Gain5/1
  Data Type Conversion4/1 -> Gain6/1
  Data Type Conversion3/1 -> Gain7/1
  Gain1/1 -> Sum/1
  Gain/1 -> Sum/2
  Gain3/1 -> Sum/3
  Gain2/1 -> Sum/4
  Gain4/1 -> Sum/5
  Gain5/1 -> Sum/6
  Gain6/1 -> Sum/7
  Gain7/1 -> Sum/8
  Digital Input/5 -> Debounce5/1
  Digital Input/6 -> Debounce6/1
  Digital Input3/1 -> Debounce4/1
  Sum/1 -> Predator Section1/1(In1)
  Digital Input4/1 -> Debounce8/1, Debounce9/1
  Debounce9/1 -> Predator Section1/Enable
  Debounce8/1 -> Predator Section/Enable
  Digital Input2/1 -> Debounce10/1
  Digital Input5/1 -> Debounce11/1
  Debounce11/1 -> Data Type Conversion9/1
  Debounce10/1 -> Data Type Conversion8/1
  Data Type Conversion8/1 -> Gain8/1
  Data Type Conversion9/1 -> Gain9/1
  Gain8/1 -> Sum/9
  Gain9/1 -> Sum/10

== system Prey_Predator_STM32F4/Predator Section/Predator Section/Predator Section/Predator Section1 ==
  In1 : Inport
  Enable : EnablePort  PropagateVarSize=During execution
  Data Store Write : DataStoreWrite  DataStoreName=D  IndexOptions=Index vector (dialog)  Indices=1  OutputSizes=1
  wires:
  In1/1 -> Data Store Write/1

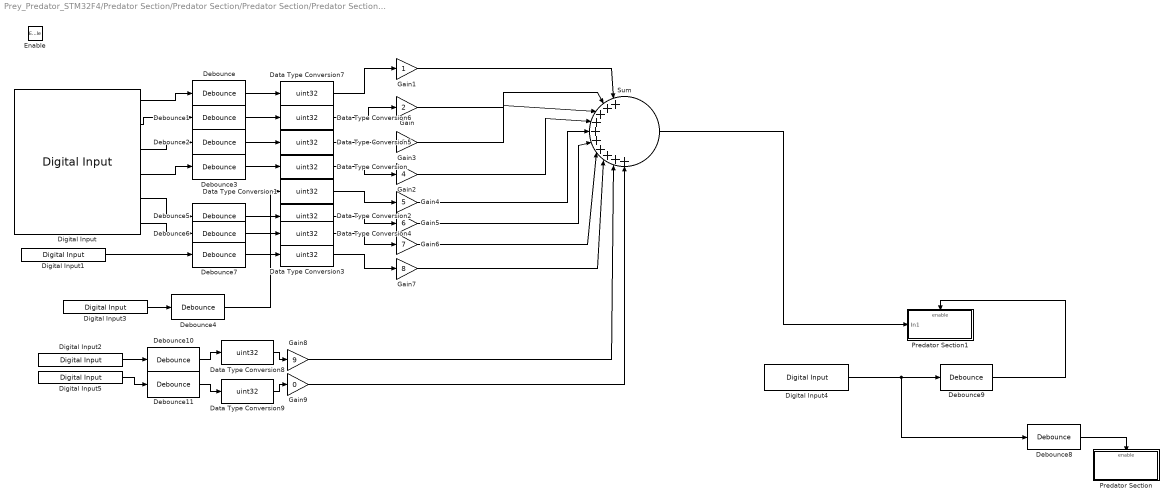
== system Prey_Predator_STM32F4/Predator Section/Predator Section/Predator Section/Predator Section/Predator Section ==
  Enable : EnablePort  PropagateVarSize=During execution
  Data Type Conversion{,1..9} (10 alike) : DataTypeConversion  OutDataTypeStr=uint32  SaturateOnIntegerOverflow=off  RndMeth=Floor
  Debounce{,1..8,10..11} (11 alike) : stm32f4_io_lib/Debounce  mode=Normal  prescale=4  debounce=4
      settings: SourceProductName=IO
  Debounce9 : stm32f4_io_lib/Debounce  mode=Single Pulse  prescale=4  debounce=4
      settings: SourceProductName=IO
  Digital Input : stm32f4_io_lib/Digital Input  port=D  speed=100  porttype=None  porttypestr=NOPULL  use_pin0=off  use_pin1=on  use_pin2=on  use_pin3=on  use_pin4=on  use_pin5=off  use_pin6=on  use_pin7=on  use_pin8=off  use_pin9=off  use_pin10=off  use_pin11=off  use_pin12=off  use_pin13=off  use_pin14=off  use_pin15=off  pinstr=GPIO_Pin_1 | GPIO_Pin_2 | GPIO_Pin_3 | GPIO_Pin_4 | GPIO_Pin_6 | GPIO_Pin_7  usedpinarray="[0  1  1  1  1  0  1  1  0  0  0  0  0  0  0  0]"  bitbandingstr=|  sampletime=0.01  sampletimestr=-1  blockid=PredatorSectionPredatorSectionPredatorSectionPredatorSectionPredatorSectionDigitalInput  enablecustomportlabel=off  glabalinit=off  cinputportlabel=In1, In2  coutputportlabel=Out1, Out2
      | #define PredatorSectionPredatorSectionPredatorSectionPredatorSectionPredatorSectionDigitalInput_D1 Peripheral_BB(GPIOD->IDR, 1)  /* Output pin */
      | #define PredatorSectionPredatorSectionPredatorSectionPredatorSectionPredatorSectionDigitalInput_D2 Peripheral_BB(GPIOD->IDR, 2)  /* Output pin */
      | #define PredatorSectionPredatorSectionPredatorSectionPredatorSectionPredatorSectionDigitalInput_D3 Peripheral_BB(GPIOD->IDR, 3)  /* Output pin */
      | #define PredatorSectionPredatorSectionPredatorSectionPredatorSectionPredatorSectionDigitalInput_D4 Peripheral_BB(GPIOD->IDR, 4)  /* Output pin */
      | #define PredatorSectionPredatorSectionPredatorSectionPredatorSectionPredatorSectionDigitalInput_D6 Peripheral_BB(GPIOD->IDR, 6)  /* Output pin */
      | #define PredatorSectionPredatorSectionPredatorSectionPredatorSectionPredatorSectionDigitalInput_D7 Peripheral_BB(GPIOD->IDR, 7)  /* Output pin */
      settings: SourceProductName=IO
  Digital Input1 : stm32f4_io_lib/Digital Input  port=B  speed=100  porttype=None  porttypestr=NOPULL  use_pin0=off  use_pin1=off  use_pin2=off  use_pin3=on  use_pin4=off  use_pin5=off  use_pin6=off  use_pin7=off  use_pin8=off  use_pin9=off  use_pin10=off  use_pin11=off  use_pin12=off  use_pin13=off  use_pin14=off  use_pin15=off  pinstr=GPIO_Pin_3  usedpinarray="[0  0  0  1  0  0  0  0  0  0  0  0  0  0  0  0]"  bitbandingstr="#define PredatorSectionPredatorSectionPredatorSectionPredatorSectionPredatorSectionDigitalInput1_B3 Peripheral_BB(GPIOB->IDR, 3)  /* Output pin */"  sampletime=0.01  sampletimestr=-1  blockid=PredatorSectionPredatorSectionPredatorSectionPredatorSectionPredatorSectionDigitalInput1  enablecustomportlabel=off  glabalinit=off  cinputportlabel=In1, In2  coutputportlabel=Out1, Out2
      settings: SourceProductName=IO
  Digital Input2 : stm32f4_io_lib/Digital Input  port=A  speed=100  porttype=None  porttypestr=NOPULL  use_pin0=off  use_pin1=on  use_pin2=off  use_pin3=off  use_pin4=off  use_pin5=off  use_pin6=off  use_pin7=off  use_pin8=off  use_pin9=off  use_pin10=off  use_pin11=off  use_pin12=off  use_pin13=off  use_pin14=off  use_pin15=off  pinstr=GPIO_Pin_1  usedpinarray="[0  1  0  0  0  0  0  0  0  0  0  0  0  0  0  0]"  bitbandingstr="#define PredatorSectionPredatorSectionPredatorSectionPredatorSectionPredatorSectionDigitalInput2_A1 Peripheral_BB(GPIOA->IDR, 1)  /* Output pin */"  sampletime=0.01  sampletimestr=-1  blockid=PredatorSectionPredatorSectionPredatorSectionPredatorSectionPredatorSectionDigitalInput2  enablecustomportlabel=off  glabalinit=off  cinputportlabel=In1, In2  coutputportlabel=Out1, Out2
      settings: SourceProductName=IO
  Digital Input3 : stm32f4_io_lib/Digital Input  port=B  speed=100  porttype=None  porttypestr=NOPULL  use_pin0=off  use_pin1=off  use_pin2=off  use_pin3=off  use_pin4=off  use_pin5=on  use_pin6=off  use_pin7=off  use_pin8=off  use_pin9=off  use_pin10=off  use_pin11=off  use_pin12=off  use_pin13=off  use_pin14=off  use_pin15=off  pinstr=GPIO_Pin_5  usedpinarray="[0  0  0  0  0  1  0  0  0  0  0  0  0  0  0  0]"  bitbandingstr="#define PredatorSectionPredatorSectionPredatorSectionPredatorSectionPredatorSectionDigitalInput3_B5 Peripheral_BB(GPIOB->IDR, 5)  /* Output pin */"  sampletime=0.01  sampletimestr=-1  blockid=PredatorSectionPredatorSectionPredatorSectionPredatorSectionPredatorSectionDigitalInput3  enablecustomportlabel=off  glabalinit=off  cinputportlabel=In1, In2  coutputportlabel=Out1, Out2
      settings: SourceProductName=IO
  Digital Input4 : stm32f4_io_lib/Digital Input  port=E  speed=100  porttype=None  porttypestr=NOPULL  use_pin0=off  use_pin1=off  use_pin2=off  use_pin3=off  use_pin4=off  use_pin5=off  use_pin6=on  use_pin7=off  use_pin8=off  use_pin9=off  use_pin10=off  use_pin11=off  use_pin12=off  use_pin13=off  use_pin14=off  use_pin15=off  pinstr=GPIO_Pin_6  usedpinarray="[0  0  0  0  0  0  1  0  0  0  0  0  0  0  0  0]"  bitbandingstr="#define PredatorSectionPredatorSectionPredatorSectionPredatorSectionPredatorSectionDigitalInput4_E6 Peripheral_BB(GPIOE->IDR, 6)  /* Output pin */"  sampletime=0.01  sampletimestr=-1  blockid=PredatorSectionPredatorSectionPredatorSectionPredatorSectionPredatorSectionDigitalInput4  enablecustomportlabel=off  glabalinit=off  cinputportlabel=In1, In2  coutputportlabel=Out1, Out2
      settings: SourceProductName=IO
  Digital Input5 : stm32f4_io_lib/Digital Input  port=A  speed=100  porttype=None  porttypestr=NOPULL  use_pin0=on  use_pin1=off  use_pin2=off  use_pin3=off  use_pin4=off  use_pin5=off  use_pin6=off  use_pin7=off  use_pin8=off  use_pin9=off  use_pin10=off  use_pin11=off  use_pin12=off  use_pin13=off  use_pin14=off  use_pin15=off  pinstr=GPIO_Pin_0  usedpinarray="[1  0  0  0  0  0  0  0  0  0  0  0  0  0  0  0]"  bitbandingstr="#define PredatorSectionPredatorSectionPredatorSectionPredatorSectionPredatorSectionDigitalInput5_A0 Peripheral_BB(GPIOA->IDR, 0)  /* Output pin */"  sampletime=0.01  sampletimestr=-1  blockid=PredatorSectionPredatorSectionPredatorSectionPredatorSectionPredatorSectionDigitalInput5  enablecustomportlabel=off  glabalinit=off  cinputportlabel=In1, In2  coutputportlabel=Out1, Out2
      settings: SourceProductName=IO
  Gain : Gain  Gain=2  OutDataTypeStr=Inherit: Same as input
  Gain1 : Gain  OutDataTypeStr=Inherit: Same as input
  Gain2 : Gain  Gain=4  OutDataTypeStr=Inherit: Same as input
  Gain3 : Gain  Gain=3  OutDataTypeStr=Inherit: Same as input
  Gain4 : Gain  Gain=5  OutDataTypeStr=Inherit: Same as input
  Gain5 : Gain  Gain=6  OutDataTypeStr=Inherit: Same as input
  Gain6 : Gain  Gain=7  OutDataTypeStr=Inherit: Same as input
  Gain7 : Gain  Gain=8  OutDataTypeStr=Inherit: Same as input
  Gain8 : Gain  Gain=9  OutDataTypeStr=Inherit: Same as input
  Gain9 : Gain  Gain=0  OutDataTypeStr=Inherit: Same as input
  Predator Section : Subsystem
  Predator Section1 : Subsystem
  Sum : Sum  Inputs=|++++++++++
  wires:
  Digital Input/4 -> Debounce3/1
  Digital Input/3 -> Debounce2/1
  Digital Input/2 -> Debounce1/1
  Digital Input/1 -> Debounce/1
  Digital Input1/1 -> Debounce7/1
  Debounce/1 -> Data Type Conversion7/1
  Debounce1/1 -> Data Type Conversion6/1
  Debounce2/1 -> Data Type Conversion5/1
  Debounce3/1 -> Data Type Conversion/1
  Debounce4/1 -> Data Type Conversion1/1
  Debounce5/1 -> Data Type Conversion2/1
  Debounce6/1 -> Data Type Conversion4/1
  Debounce7/1 -> Data Type Conversion3/1
  Data Type Conversion7/1 -> Gain1/1
  Data Type Conversion6/1 -> Gain/1
  Data Type Conversion5/1 -> Gain3/1
  Data Type Conversion/1 -> Gain2/1
  Data Type Conversion1/1 -> Gain4/1
  Data Type Conversion2/1 -> Gain5/1
  Data Type Conversion4/1 -> Gain6/1
  Data Type Conversion3/1 -> Gain7/1
  Gain1/1 -> Sum/1
  Gain/1 -> Sum/2
  Gain3/1 -> Sum/3
  Gain2/1 -> Sum/4
  Gain4/1 -> Sum/5
  Gain5/1 -> Sum/6
  Gain6/1 -> Sum/7
  Gain7/1 -> Sum/8
  Digital Input/5 -> Debounce5/1
  Digital Input/6 -> Debounce6/1
  Digital Input3/1 -> Debounce4/1
  Sum/1 -> Predator Section1/1(In1)
  Digital Input4/1 -> Debounce8/1, Debounce9/1
  Debounce9/1 -> Predator Section1/Enable
  Debounce8/1 -> Predator Section/Enable
  Digital Input2/1 -> Debounce10/1
  Digital Input5/1 -> Debounce11/1
  Debounce11/1 -> Data Type Conversion9/1
  Debounce10/1 -> Data Type Conversion8/1
  Data Type Conversion8/1 -> Gain8/1
  Data Type Conversion9/1 -> Gain9/1
  Gain8/1 -> Sum/9
  Gain9/1 -> Sum/10

== system Prey_Predator_STM32F4/Predator Section/Predator Section/Predator Section/Predator Section/Predator Section1 ==
  In1 : Inport
  Enable : EnablePort  PropagateVarSize=During execution
  Data Store Write : DataStoreWrite  DataStoreName=E  IndexOptions=Index vector (dialog)  Indices=1  OutputSizes=1
  wires:
  In1/1 -> Data Store Write/1
